simulink model "CO2control"  (R2025a)
settings: Solver=VariableStepAuto  StartTime=0.0  StopTime=2000.0  RelTol=1e-3
settings Model: Creator=Laurenpearse  LastModifiedBy=Laurenpearse

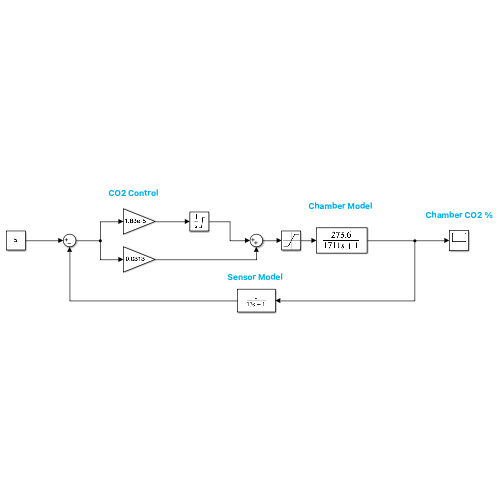
[thumbnail: Simulink's stored preview of the top-level diagram]
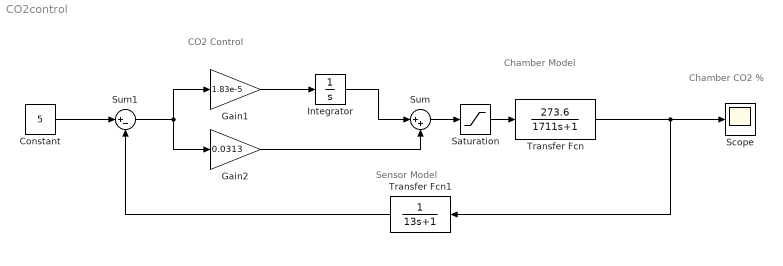
== system CO2control ==
  note: CO2 Control
  note: Chamber Model
  note: Sensor Model
  note: Chamber CO2 %
  Constant : Constant  Value=5
  Gain1 : Gain  Gain=1.83e-5
  Gain2 : Gain  Gain=0.0313
  Integrator : Integrator  LimitOutput=on  UpperSaturationLimit=1  LowerSaturationLimit=0
  Saturation : Saturate  UpperLimit=1  LowerLimit=0
  Scope : Scope
      settings: ActiveDisplayYMinimum=-0.62499700024211868  ActiveDisplayYMaximum=5.6249730021790691
  Sum : Sum  Inputs=|++
  Sum1 : Sum  Inputs=|+-
  Transfer Fcn : TransferFcn  Numerator=273.6  Denominator=[1711 1]
  Transfer Fcn1 : TransferFcn  Denominator="[13  1]"
  wires:
  Gain1/1 -> Integrator/1
  Integrator/1 -> Sum/1
  Gain2/1 -> Sum/2
  Sum/1 -> Saturation/1
  Transfer Fcn/1 -> Transfer Fcn1/1, Scope/1
  Constant/1 -> Sum1/1
  Sum1/1 -> Gain2/1, Gain1/1
  Saturation/1 -> Transfer Fcn/1
  Transfer Fcn1/1 -> Sum1/2
